simulink model "EV_charging_V2G_and_G2V"  (R2024b)
settings: Solver=ode23t  StartTime=0.0  StopTime=1  RelTol=1e-3
undefined symbols (not defined in the file): Ion, Lithium
libraries: spsSeriesRLCBranchLib x8, spsIGBTDiodeLib x4, slpidlib x2, spsCurrentMeasurementLib x2, spsMosfetLib x2, spsVoltageMeasurementLib x2, spsACVoltageSourceLib x1, spsBatteryLib x1, spsPLLLib x1, spsPWMGenerator2LevelLib x1, spsPWMGeneratorDCDCLib x1, sps_lib x1
settings Model: Creator=SUDHAK1  LastModifiedBy=SUDHAK1

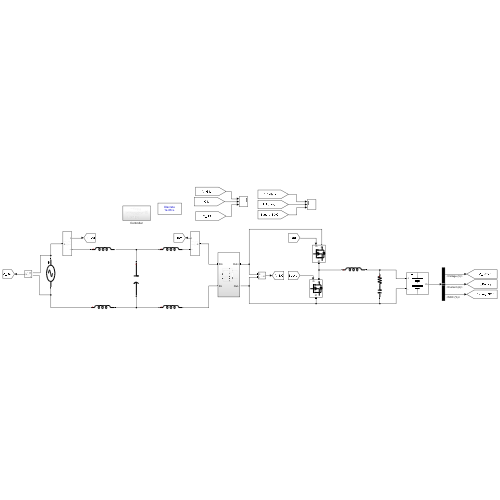
[thumbnail: Simulink's stored preview of the top-level diagram]
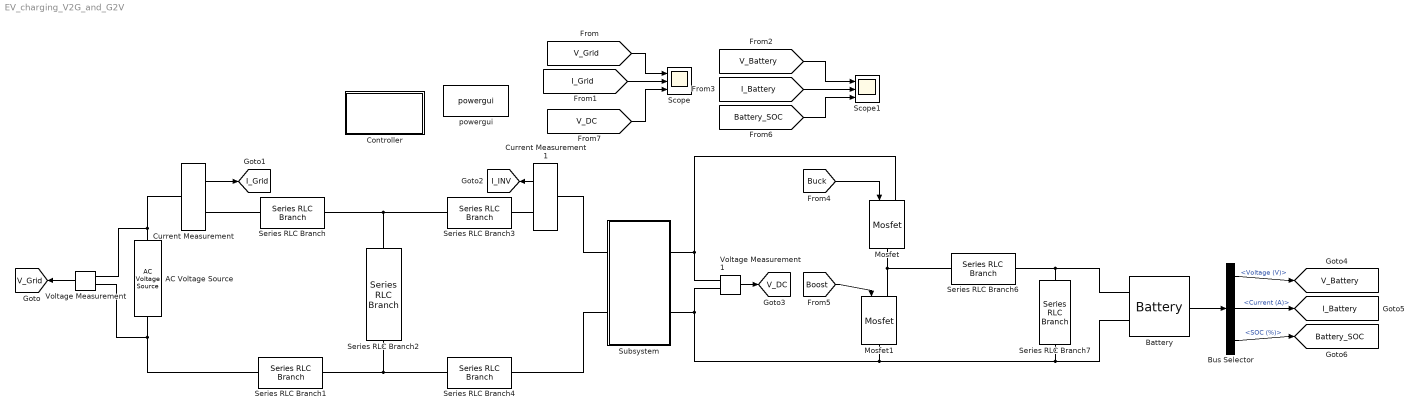
== system EV_charging_V2G_and_G2V ==
  AC Voltage Source : spsACVoltageSourceLib/AC Voltage Source  Amplitude=325  Phase=0  Frequency=50  SampleTime=0  Measurements=None  BusType=swing  Pref=10e3  Qref=0  Qmin=-inf  Qmax=+inf
  Battery : spsBatteryLib/Battery  BatType=Lithium-Ion  NomV=160  NomQ=120  SOC=50  Batt_Tr=1  PresetModel=on  MaxQ=120  MinV=120  FullV=186.2379  Dis_rate=52.1739  R=0.013333  Normal_OP=108.5217  expZone="[172.8617      5.895652]"
  Bus Selector : BusSelector  OutputSignals=Voltage (V),Current (A),SOC (%)
  Controller : Subsystem
  Current Measurement : spsCurrentMeasurementLib/Current Measurement  PhasorSimulation=off  OutputType=Complex  PSBequivalent=0
  Current Measurement1 : spsCurrentMeasurementLib/Current Measurement  PhasorSimulation=off  OutputType=Complex  PSBequivalent=0
  Mosfet : spsMosfetLib/Mosfet  Ron=0.1  Lon=0  Rd=0.01  Vfd=0  IC=0  Rs=1e5  Cs=inf  Measurements=off
  Mosfet1 : spsMosfetLib/Mosfet  Ron=0.1  Lon=0  Rd=0.01  Vfd=0  IC=0  Rs=1e5  Cs=inf  Measurements=off
  Scope : Scope  NumInputPorts=3
  Scope1 : Scope  NumInputPorts=3
  Series RLC Branch : spsSeriesRLCBranchLib/Series RLC Branch  LConnTagsString=__new0  RConnTagsString=__new0  BranchType=L  Resistance=1  Inductance=2.18e-3  SetiL0=off  InitialCurrent=0  Capacitance=1e-6  Setx0=off  InitialVoltage=0  Measurements=None
  Series RLC Branch1 : spsSeriesRLCBranchLib/Series RLC Branch  LConnTagsString=__new0  RConnTagsString=__new0  BranchType=L  Resistance=1  Inductance=2.18e-3  SetiL0=off  InitialCurrent=0  Capacitance=1e-6  Setx0=off  InitialVoltage=0  Measurements=None
  Series RLC Branch2 : spsSeriesRLCBranchLib/Series RLC Branch  LConnTagsString=__new0  RConnTagsString=__new0  BranchType=C  Resistance=1  Inductance=2.18e-3  SetiL0=off  InitialCurrent=0  Capacitance=6.23e-6  Setx0=off  InitialVoltage=0  Measurements=None
  Series RLC Branch3 : spsSeriesRLCBranchLib/Series RLC Branch  LConnTagsString=__new0  RConnTagsString=__new0  BranchType=L  Resistance=1  Inductance=2.03e-3  SetiL0=off  InitialCurrent=0  Capacitance=1e-6  Setx0=off  InitialVoltage=0  Measurements=None
  Series RLC Branch4 : spsSeriesRLCBranchLib/Series RLC Branch  LConnTagsString=__new0  RConnTagsString=__new0  BranchType=L  Resistance=1  Inductance=2.03e-3  SetiL0=off  InitialCurrent=0  Capacitance=1e-6  Setx0=off  InitialVoltage=0  Measurements=None
  Series RLC Branch6 : spsSeriesRLCBranchLib/Series RLC Branch  LConnTagsString=__new0  RConnTagsString=__new0  BranchType=L  Resistance=0.0001  Inductance=20e-3  SetiL0=off  InitialCurrent=0  Capacitance=5600e-6  Setx0=on  InitialVoltage=400  Measurements=None
  Series RLC Branch7 : spsSeriesRLCBranchLib/Series RLC Branch  LConnTagsString=__new0  RConnTagsString=__new0  BranchType=RC  Resistance=0.0001  Inductance=20e-3  SetiL0=off  InitialCurrent=0  Capacitance=100e-6  Setx0=off  InitialVoltage=400  Measurements=None
  Subsystem : Subsystem
  Voltage Measurement : spsVoltageMeasurementLib/Voltage Measurement  PhasorSimulation=off  OutputType=Complex  PSBequivalent=0
  Voltage Measurement1 : spsVoltageMeasurementLib/Voltage Measurement  PhasorSimulation=off  OutputType=Complex  PSBequivalent=0
  powergui : sps_lib/powergui  Priority=1  SimulationMode=Discrete  SampleTime=1e-6  frequency=60  Iterations=50  frequencyindice=50  Pbase=100e6  ErrMax=1e-4  UnitsV=kV  UnitsW=MW  buscounter=0  FunctionMessages=off  echomessages=off  EnableUseOfTLC=off  CurrentSourceSwitches=off  DisableSnubberDevices=off  DisableRonSwitches=off  DisableVfSwitches=off  DisplayEquations=off  AutomaticDiscreteSolvers=off  SolverType=Tustin/Backward Euler (TBE)  Interpol=off  ExternalGateDelay=off  methode=off  Ts=100  x0status=blocks  SPID=on  SwTol=0  HookPort=off  NonlinearTolerance=1e-4  nMaxIteration=100  ContinueOnMaxIteration=off  RestoreLinks=warning  ResistiveCurrentMeasurement=off  Frange=[0:2:500]  Ylog=off  Xlog=on  ShowGrid=off  save=off  variable=ZData  structure=0  ZoomFFT=off  StartTime=0.0  cycles=1  DisplayStyle=1  fundamental=60  FreqAxis=off  MaxFrequency=1000  frequencyindicesteady=1  RmsSteady=1  display=off
  tag scope: Battery_SOC=global, I_Battery=global, I_Grid=global, I_INV=global, V_Battery=global, V_DC=global, V_Grid=global
  wires:
  Voltage Measurement/1 -> [V_Grid]
  Current Measurement/1 -> [I_Grid]
  Voltage Measurement1/1 -> [V_DC]
  Battery/1 -> Bus Selector/1
  Bus Selector/1 -> [V_Battery]  "<Voltage (V)>"
  Bus Selector/2 -> [I_Battery]  "<Current (A)>"
  Bus Selector/3 -> [Battery_SOC]  "<SOC (%)>"
  Current Measurement1/1 -> [I_INV]
  [Boost] -> Mosfet1/1
  [Buck] -> Mosfet/1
  [V_Grid] -> Scope/1
  [I_Grid] -> Scope/2
  [V_Battery] -> Scope1/1
  [I_Battery] -> Scope1/2
  [Battery_SOC] -> Scope1/3
  [V_DC] -> Scope/3
  connections:
  Current Measurement/RConn1 -- Series RLC Branch/LConn1
  Voltage Measurement/LConn1 -- Current Measurement/LConn1 -- AC Voltage Source/RConn1
  AC Voltage Source/LConn1 -- Series RLC Branch1/LConn1 -- Voltage Measurement/LConn2
  Series RLC Branch2/LConn1 -- Series RLC Branch/RConn1 -- Series RLC Branch3/LConn1
  Series RLC Branch1/RConn1 -- Series RLC Branch2/RConn1 -- Series RLC Branch4/LConn1
  Current Measurement1/RConn1 -- Series RLC Branch3/RConn1
  Current Measurement1/LConn1 -- Subsystem/LConn1
  Series RLC Branch4/RConn1 -- Subsystem/LConn2
  Voltage Measurement1/LConn1 -- Subsystem/RConn1 -- Mosfet/LConn1
  Mosfet1/RConn1 -- Series RLC Branch7/RConn1 -- Battery/LConn2 -- Subsystem/RConn2 -- Voltage Measurement1/LConn2
  Mosfet/RConn1 -- Series RLC Branch6/LConn1 -- Mosfet1/LConn1
  Series RLC Branch7/LConn1 -- Battery/LConn1 -- Series RLC Branch6/RConn1

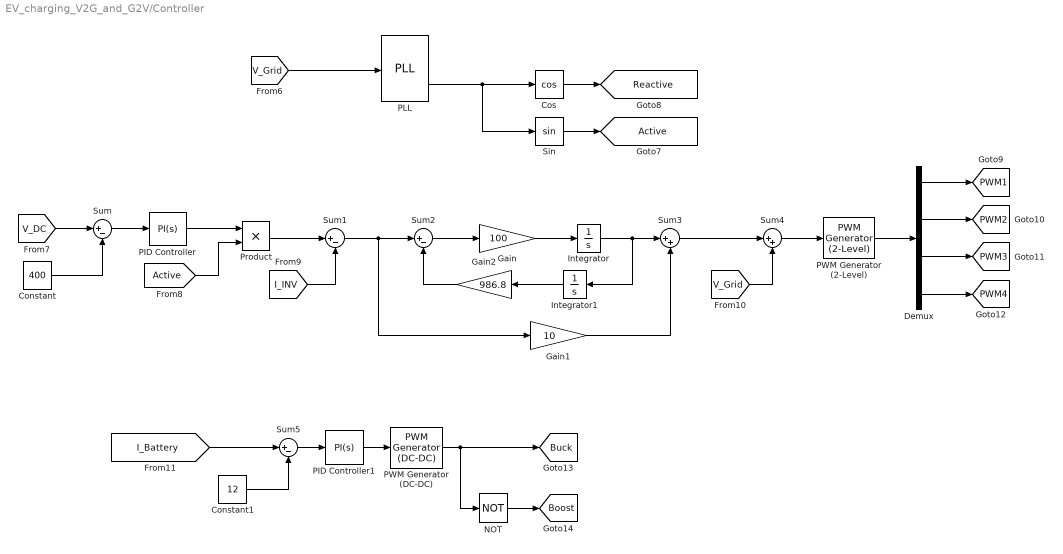
== system EV_charging_V2G_and_G2V/Controller ==
  Constant : Constant  Value=400
  Constant1 : Constant  Value=12
  Cos : Trigonometry  Operator=cos
  Demux : Demux
  Gain : Gain  Gain=100
  Gain1 : Gain  Gain=10
  Gain2 : Gain  Gain=986.8
  Integrator : Integrator
  Integrator1 : Integrator
  NOT : Logic  Operator=NOT  IconShape=distinctive  AllPortsSameDT=off  OutDataTypeStr=boolean
  PID Controller : slpidlib/PID Controller  Controller=PI  Form=Parallel  TimeDomain=Continuous-time  UseExternalTs=off  SampleTime=-1  IntegratorMethod=Forward Euler  FilterMethod=Forward Euler  ControllerParametersSource=internal  P=1  I=10  UseKiTs=off  D=0  UseExternalDerivativeSource=off  N=100  UseFilter=on  TunerSelectOption=Transfer Function Based (PID Tuner App)  InitialConditionSource=internal  InitialConditionForIntegrator=0  InitialConditionForFilter=0  DifferentiatorICPrevScaledInput=0  ExternalReset=none  TrackingMode=off  Kt=1  LimitOutput=off  SatLimitsSource=internal  UpperSaturationLimit=inf  LowerSaturationLimit=-inf  LinearizeAsGain=on  AntiWindupMode=none  Kb=1  LimitIntegrator=off  UpperIntegratorSaturationLimit=inf  LowerIntegratorSaturationLimit=-inf  POutMin=[]  POutMax=[]  IOutMin=[]  IOutMax=[]  DOutMin=[]  DOutMax=[]  NOutMin=[]  NOutMax=[]  SumOutMin=[]  SumOutMax=[]  SaturationOutMin=[]  SaturationOutMax=[]  PParamMin=[]  PParamMax=[]  IParamMin=[]  IParamMax=[]  DParamMin=[]  DParamMax=[]  NParamMin=[]  NParamMax=[]  KbParamMin=[]  KbParamMax=[]  KtParamMin=[]  KtParamMax=[]  KbOutMin=[]  KbOutMax=[]  KtOutMin=[]  KtOutMax=[]  IntegratorOutMin=[]  IntegratorOutMax=[]  FilterOutMin=[]  FilterOutMax=[]  SumI1OutMin=[]  SumI1OutMax=[]  SumI2OutMin=[]  SumI2OutMax=[]  SumI3OutMin=[]  SumI3OutMax=[]  SumI4OutMin=[]  SumI4OutMax=[]  SumDOutMin=[]  SumDOutMax=[]  DifferentiatorOutMin=[]  DifferentiatorOutMax=[]  FilterDiffOutCoefMin=[]  FilterDiffOutCoefMax=[]  ReciprocalOutMin=[]  ReciprocalOutMax=[]  SumDenOutMin=[]  SumDenOutMax=[]  SumNumOutMin=[]  SumNumOutMax=[]  DivideOutMin=[]  DivideOutMax=[]  UdiffTsProdOutMin=[]  UdiffTsProdOutMax=[]  NTsProdOutMin=[]  NTsProdOutMax=[]  UintegralTsProdOutMin=[]  UintegralTsProdOutMax=[]  UngainTsProdOutMin=[]  UngainTsProdOutMax=[]  ClampingZeroOutDataTypeStr=Inherit: Inherit via back propagation  ClampingZeroOutMin=[]  ClampingZeroOutMax=[]  FilterDenConstantOutDataTypeStr=Inherit: Inherit via back propagation  FilterDenConstantOutMin=[]  FilterDenConstantOutMax=[]  PCopyOutDataTypeStr=Inherit: Inherit via back propagation  PCopyOutMin=[]  PCopyOutMax=[]  NCopyOutDataTypeStr=Inherit: Inherit via back propagation  NCopyOutMin=[]  NCopyOutMax=[]  IntegratorContinuousStateAttributes=''  IntegratorStateMustResolveToSignalObject=off  IntegratorRTWStateStorageClass=Auto  FilterContinuousStateAttributes=''  FilterStateMustResolveToSignalObject=off  FilterRTWStateStorageClass=Auto  ParallelPVariant=InternalParameters  IdealPVariant=Disabled  IVariant=InternalParameters  DVariant=Disabled  IntegratorVariant=Continuous  SatVariant=Disabled  AWVariant=Passthrough  PCopyVariant=Disabled  TRVariant=Disabled  FdbkBlocksVariant=Forward  IdealPFdbkVariant=Disabled  SatFdbkVariant=Disabled  DerivativeFilterVariant=Disabled  NVariant=Disabled  NCopyVariant=Disabled_SignalSpec  FilterICVariant=Disabled  IntegratorICVariant=InternalICs  ExternalResetVariant=Disabled  TRSumVariant=Passthrough  SumFdbkVariant=Disabled  SumVariant=Sum_PI  TsampFilterVariant=InternalTs  TsampNgainVariant=Passthrough  TsampIntegralVariant=Disabled_SignalSpec  ExternalSaturationOutDataTypeStr=Inherit: Same as second input  DerivativeSourceVariant=Disabled  PreIntVariant=InternalPreInt
  PID Controller1 : slpidlib/PID Controller  Controller=PI  Form=Parallel  TimeDomain=Continuous-time  UseExternalTs=off  SampleTime=-1  IntegratorMethod=Forward Euler  FilterMethod=Forward Euler  ControllerParametersSource=internal  P=0.005  I=10  UseKiTs=off  D=0  UseExternalDerivativeSource=off  N=100  UseFilter=on  TunerSelectOption=Transfer Function Based (PID Tuner App)  InitialConditionSource=internal  InitialConditionForIntegrator=0  InitialConditionForFilter=0  DifferentiatorICPrevScaledInput=0  ExternalReset=none  TrackingMode=off  Kt=1  LimitOutput=on  SatLimitsSource=internal  UpperSaturationLimit=0.95  LowerSaturationLimit=0  LinearizeAsGain=on  AntiWindupMode=none  Kb=1  LimitIntegrator=off  UpperIntegratorSaturationLimit=inf  LowerIntegratorSaturationLimit=-inf  POutMin=[]  POutMax=[]  IOutMin=[]  IOutMax=[]  DOutMin=[]  DOutMax=[]  NOutMin=[]  NOutMax=[]  SumOutMin=[]  SumOutMax=[]  SaturationOutMin=[]  SaturationOutMax=[]  PParamMin=[]  PParamMax=[]  IParamMin=[]  IParamMax=[]  DParamMin=[]  DParamMax=[]  NParamMin=[]  NParamMax=[]  KbParamMin=[]  KbParamMax=[]  KtParamMin=[]  KtParamMax=[]  KbOutMin=[]  KbOutMax=[]  KtOutMin=[]  KtOutMax=[]  IntegratorOutMin=[]  IntegratorOutMax=[]  FilterOutMin=[]  FilterOutMax=[]  SumI1OutMin=[]  SumI1OutMax=[]  SumI2OutMin=[]  SumI2OutMax=[]  SumI3OutMin=[]  SumI3OutMax=[]  SumI4OutMin=[]  SumI4OutMax=[]  SumDOutMin=[]  SumDOutMax=[]  DifferentiatorOutMin=[]  DifferentiatorOutMax=[]  FilterDiffOutCoefMin=[]  FilterDiffOutCoefMax=[]  ReciprocalOutMin=[]  ReciprocalOutMax=[]  SumDenOutMin=[]  SumDenOutMax=[]  SumNumOutMin=[]  SumNumOutMax=[]  DivideOutMin=[]  DivideOutMax=[]  UdiffTsProdOutMin=[]  UdiffTsProdOutMax=[]  NTsProdOutMin=[]  NTsProdOutMax=[]  UintegralTsProdOutMin=[]  UintegralTsProdOutMax=[]  UngainTsProdOutMin=[]  UngainTsProdOutMax=[]  ClampingZeroOutDataTypeStr=Inherit: Inherit via back propagation  ClampingZeroOutMin=[]  ClampingZeroOutMax=[]  FilterDenConstantOutDataTypeStr=Inherit: Inherit via back propagation  FilterDenConstantOutMin=[]  FilterDenConstantOutMax=[]  PCopyOutDataTypeStr=Inherit: Inherit via back propagation  PCopyOutMin=[]  PCopyOutMax=[]  NCopyOutDataTypeStr=Inherit: Inherit via back propagation  NCopyOutMin=[]  NCopyOutMax=[]  IntegratorContinuousStateAttributes=''  IntegratorStateMustResolveToSignalObject=off  IntegratorRTWStateStorageClass=Auto  FilterContinuousStateAttributes=''  FilterStateMustResolveToSignalObject=off  FilterRTWStateStorageClass=Auto  ParallelPVariant=InternalParameters  IdealPVariant=Disabled  IVariant=InternalParameters  DVariant=Disabled  IntegratorVariant=Continuous  SatVariant=Enabled  AWVariant=Passthrough  PCopyVariant=Disabled  TRVariant=Disabled  FdbkBlocksVariant=Forward  IdealPFdbkVariant=Disabled  SatFdbkVariant=Disabled  DerivativeFilterVariant=Disabled  NVariant=Disabled  NCopyVariant=Disabled_SignalSpec  FilterICVariant=Disabled  IntegratorICVariant=InternalICs  ExternalResetVariant=Disabled  TRSumVariant=Passthrough  SumFdbkVariant=Disabled  SumVariant=Sum_PI  TsampFilterVariant=InternalTs  TsampNgainVariant=Passthrough  TsampIntegralVariant=Disabled_SignalSpec  ExternalSaturationOutDataTypeStr=Inherit: Same as second input  DerivativeSourceVariant=Disabled  PreIntVariant=InternalPreInt
  PLL : spsPLLLib/PLL  Fmin=45  Par_Init=[0, 50]  ParK=[180, 3200, 1]  TcD=1e-6  MaxRateChangeFreq=12  FilterCutOffFreq=25  Ts=0  AGC=on
      settings: LibrarySourceBlock=sps_lib/Control/PLL
  PWM Generator (2-Level) : spsPWMGenerator2LevelLib/PWM Generator (2-Level)  ModulatorType=Single-phase full-bridge (4 pulses)  ModulatorMode=Unsynchronized  Fc=10000  Pc=90  nF=27  MinMax="[ -1  1 ]"  SamplingTechnique=Natural  ModulatingSignals=off  m=0.8  Freq=60  Phase=0  Ts=0  ShowCarrierOutport=off
  PWM Generator (DC-DC) : spsPWMGeneratorDCDCLib/PWM Generator (DC-DC)  Fsw=10000  Ts=0
  Product : Product
  Sin : Trigonometry
  Sum{,1..2,5} (4 alike) : Sum  Inputs=|+-
  Sum3 : Sum  Inputs=|++
  Sum4 : Sum  Inputs=|++
  tag scope: Active=global, Boost=global, Buck=global, PWM1=global, PWM2=global, PWM3=global, PWM4=global, Reactive=global
  wires:
  Sum1/1 -> Gain1/1, Sum2/1
  Product/1 -> Sum1/1
  Sum4/1 -> PWM Generator (2-Level)/1
  Integrator/1 -> Integrator1/1, Sum3/1
  Integrator1/1 -> Gain2/1
  Constant/1 -> Sum/2
  Demux/4 -> [PWM4]
  PWM Generator (DC-DC)/1 -> NOT/1, [Buck]
  PWM Generator (2-Level)/1 -> Demux/1
  Sum5/1 -> PID Controller1/1
  Demux/2 -> [PWM2]
  Constant1/1 -> Sum5/2
  PID Controller1/1 -> PWM Generator (DC-DC)/1
  Sum3/1 -> Sum4/1
  Sum/1 -> PID Controller/1
  NOT/1 -> [Boost]
  Gain/1 -> Integrator/1
  Gain1/1 -> Sum3/2
  [V_Grid] -> Sum4/2
  [V_DC] -> Sum/1
  Demux/1 -> [PWM1]
  Gain2/1 -> Sum2/2
  Demux/3 -> [PWM3]
  Sum2/1 -> Gain/1
  PID Controller/1 -> Product/1
  [I_INV] -> Sum1/2
  [I_Battery] -> Sum5/1
  [Active] -> Product/2
  Cos/1 -> [Reactive]
  [V_Grid] -> PLL/1
  Sin/1 -> [Active]
  PLL/2 -> Cos/1, Sin/1

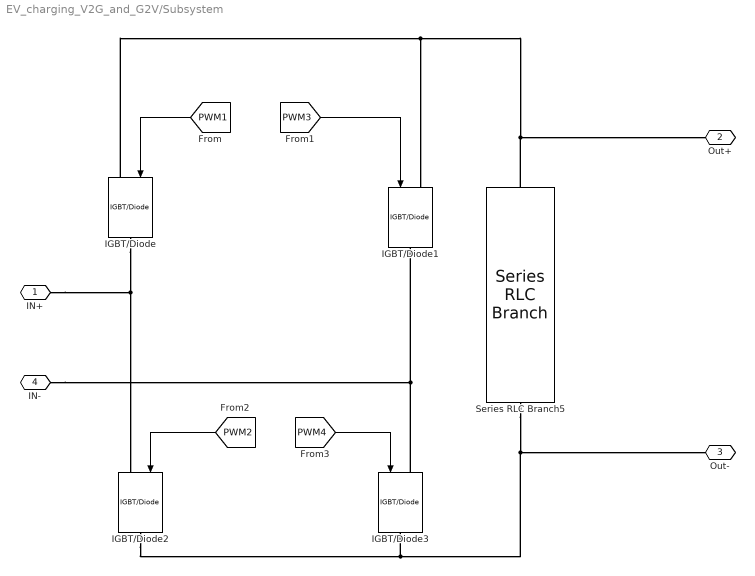
== system EV_charging_V2G_and_G2V/Subsystem ==
  IGBT/Diode{,1..3} (4 alike) : spsIGBTDiodeLib/IGBT//Diode  Ron=1e-3  Rs=1e5  Cs=inf  Measurements=off
  Series RLC Branch5 : spsSeriesRLCBranchLib/Series RLC Branch  LConnTagsString=__new0  RConnTagsString=__new0  BranchType=RC  Resistance=0.0001  Inductance=2.03e-3  SetiL0=off  InitialCurrent=0  Capacitance=5600e-6  Setx0=on  InitialVoltage=400  Measurements=None
  IN+ : PMIOPort  Side=Left
  Out+ : PMIOPort  Port=2  Side=Right
  Out- : PMIOPort  Port=3  Side=Right
  IN- : PMIOPort  Port=4  Side=Left
  wires:
  [PWM1] -> IGBT/Diode/1
  [PWM2] -> IGBT/Diode2/1
  [PWM3] -> IGBT/Diode1/1
  [PWM4] -> IGBT/Diode3/1
  connections:
  IGBT/Diode3/LConn1 -- IN-/RConn1 -- IGBT/Diode1/RConn1
  IGBT/Diode2/RConn1 -- IGBT/Diode3/RConn1 -- Series RLC Branch5/RConn1 -- Out-/RConn1
  IGBT/Diode/LConn1 -- IGBT/Diode1/LConn1 -- Series RLC Branch5/LConn1 -- Out+/RConn1
  IGBT/Diode/RConn1 -- IN+/RConn1 -- IGBT/Diode2/LConn1
